simulink model "pvwindupfc11"  (R2016a)
settings: Solver=VariableStepAuto  StartTime=0.0  StopTime=0.5  RelTol=1e-3
undefined symbols (not defined in the file): BCMS11, c1, c2, c3, c4, c5, c6, Clink_3L, DiscIntNeverNeededParam, fdesignblkfcn, Fnom, gcbh, Ion, Ki_Ireg_3L, Ki_VDCreg_3L, Kp_Ireg_3L, Kp_VDCreg_3L, LimitL_Ireg_3L, LimitL_VDCreg_3L, LimitU_Ireg_3L, LimitU_VDCreg_3L, Lithium, LowerLimit, Pnom_3L, Pnom_dc_3L, PV11, Ts_Control, Ts_Power, Ts_PWM, UpperLimit, Vnom_dc_3L, Vnom_prim_3L, Vnom_sec_3L
libraries: powerlib x98, powerlib_extras x29, powerlib_meascontrol x20, fuzblock x2, simulink x1, electricdrivelib x1
(part 4 of 4)

== system pvwindupfc11/Control Systems /SEC Control/SEC Control System/Scaling ==
  Vdc : Inport
  VdVq : Inport  Port=2
  0.8 to 1.2 x Vnom_dc : Saturate  UpperLimit=1.5*Vnom_dc_3L  LowerLimit=0.5*Vnom_dc_3L
  Constant1 : Constant  Value=Vnom_sec_3L
  Gain1 : Gain  Gain=0.5/sqrt(2)*sqrt(3)
  Product : Product  Inputs=*/
  Product1 : Product  Inputs=**
  VdVq* : Outport
  wires:
  Product1/1 -> VdVq*/1
  VdVq/1 -> Product1/1
  Vdc/1 -> 0.8 to 1.2 x Vnom_dc/1
  Product/1 -> Product1/2
  0.8 to 1.2 x Vnom_dc/1 -> Gain1/1
  Gain1/1 -> Product/2
  Constant1/1 -> Product/1

== system pvwindupfc11/Control Systems /SEC Control/SEC Control System/VDC Controller ==
  Vdc : Inport  PortDimensions=1
  Vdc_ref : Inport  Port=2  PortDimensions=1
  Gain : Gain  Gain=1/(Vnom_dc_3L)
  PI_d : Subsystem  DialogController=POWERSYS.PowerSysDialog  mask(Discrete PI Controller){Kp=Kp_VDCreg_3L, Ki=Ki_VDCreg_3L, Par_Limits=[ LimitU_VDCreg_3L LimitL_VDCreg_3L ], Init=0, Ts=Ts_Control}
      mask prompts: Kp "Proportional gain (Kp):"; Ki "Integral gain (Ki):"; Par_Limits "Output limits: [ Upper   Lower ]"; Init "Output initial value:"; Ts "Sample time:"
      mask help: This block implements a discrete PI controller.
      mask init:
      | UpperLimit=Par_Limits(1);
      | LowerLimit=Par_Limits(2);
      mask Display: disp('PI');
  Sum : Sum  Inputs=|+-
  Idref : Outport
  wires:
  PI_d/1(Out) -> Idref/1
  Gain/1 -> PI_d/1(Error)
  Vdc/1 -> Sum/2
  Vdc_ref/1 -> Sum/1
  Sum/1 -> Gain/1

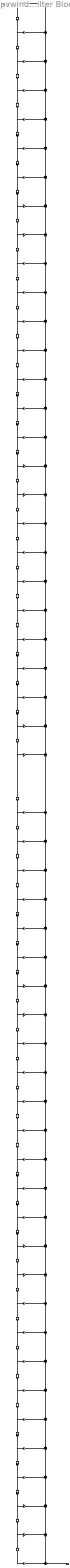
== system pvwindupfc11/Wind-MPPT/Torque reference 1/Differentiator Filter/Generated Filter Block ==
  Input : Inport
  BodyDelay{2..27,30..55} (52 alike) : Delay  DelayLength=1  InitialCondition=0  InputProcessing=Inherited
  BodyDelay29 : Delay  InitialCondition=0  InputProcessing=Inherited
  BodyLSum{2..27,29..55} (53 alike) : Sum  Inputs=++|  SaturateOnIntegerOverflow=on  InputSameDT=on  OutDataTypeStr=Inherit: Same as first input
  b(1) : Gain  Gain=0.0016485839041717864  SaturateOnIntegerOverflow=on  OutDataTypeStr=Inherit: Same as input  ParamDataTypeStr=Inherit: Same as input
  b(10) : Gain  Gain=0.011014879869749052  SaturateOnIntegerOverflow=on  OutDataTypeStr=Inherit: Same as input  ParamDataTypeStr=Inherit: Same as input
  b(11) : Gain  Gain=-0.005763535930488302  SaturateOnIntegerOverflow=on  OutDataTypeStr=Inherit: Same as input  ParamDataTypeStr=Inherit: Same as input
  b(12) : Gain  Gain=-0.0151981830555213  SaturateOnIntegerOverflow=on  OutDataTypeStr=Inherit: Same as input  ParamDataTypeStr=Inherit: Same as input
  b(13) : Gain  Gain=0.0065686388642668125  SaturateOnIntegerOverflow=on  OutDataTypeStr=Inherit: Same as input  ParamDataTypeStr=Inherit: Same as input
  b(14) : Gain  Gain=0.020867949959447688  SaturateOnIntegerOverflow=on  OutDataTypeStr=Inherit: Same as input  ParamDataTypeStr=Inherit: Same as input
  b(15) : Gain  Gain=-0.0070602627960907726  SaturateOnIntegerOverflow=on  OutDataTypeStr=Inherit: Same as input  ParamDataTypeStr=Inherit: Same as input
  b(16) : Gain  Gain=-0.028242635943863115  SaturateOnIntegerOverflow=on  OutDataTypeStr=Inherit: Same as input  ParamDataTypeStr=Inherit: Same as input
  b(17) : Gain  Gain=0.0072704924773104732  SaturateOnIntegerOverflow=on  OutDataTypeStr=Inherit: Same as input  ParamDataTypeStr=Inherit: Same as input
  b(18) : Gain  Gain=0.038329320446368831  SaturateOnIntegerOverflow=on  OutDataTypeStr=Inherit: Same as input  ParamDataTypeStr=Inherit: Same as input
  b(19) : Gain  Gain=-0.0068002265270407491  SaturateOnIntegerOverflow=on  OutDataTypeStr=Inherit: Same as input  ParamDataTypeStr=Inherit: Same as input
  b(2) : Gain  Gain=0.00017042943589110223  SaturateOnIntegerOverflow=on  OutDataTypeStr=Inherit: Same as input  ParamDataTypeStr=Inherit: Same as input
  b(20) : Gain  Gain=-0.052819993002155965  SaturateOnIntegerOverflow=on  OutDataTypeStr=Inherit: Same as input  ParamDataTypeStr=Inherit: Same as input
  b(21) : Gain  Gain=0.0049482783503700268  SaturateOnIntegerOverflow=on  OutDataTypeStr=Inherit: Same as input  ParamDataTypeStr=Inherit: Same as input
  b(22) : Gain  Gain=0.075871674298216826  SaturateOnIntegerOverflow=on  OutDataTypeStr=Inherit: Same as input  ParamDataTypeStr=Inherit: Same as input
  b(23) : Gain  Gain=0.00073312852370662537  SaturateOnIntegerOverflow=on  OutDataTypeStr=Inherit: Same as input  ParamDataTypeStr=Inherit: Same as input
  b(24) : Gain  Gain=-0.11992357305817197  SaturateOnIntegerOverflow=on  OutDataTypeStr=Inherit: Same as input  ParamDataTypeStr=Inherit: Same as input
  b(25) : Gain  Gain=-0.022982436984387535  SaturateOnIntegerOverflow=on  OutDataTypeStr=Inherit: Same as input  ParamDataTypeStr=Inherit: Same as input
  b(26) : Gain  Gain=0.24743192698089667  SaturateOnIntegerOverflow=on  OutDataTypeStr=Inherit: Same as input  ParamDataTypeStr=Inherit: Same as input
  b(27) : Gain  Gain=0.30572927022108953  SaturateOnIntegerOverflow=on  OutDataTypeStr=Inherit: Same as input  ParamDataTypeStr=Inherit: Same as input
  b(29) : Gain  Gain=-0.30572927022108953  SaturateOnIntegerOverflow=on  OutDataTypeStr=Inherit: Same as input  ParamDataTypeStr=Inherit: Same as input
  b(3) : Gain  Gain=-0.0038948238157296179  SaturateOnIntegerOverflow=on  OutDataTypeStr=Inherit: Same as input  ParamDataTypeStr=Inherit: Same as input
  b(30) : Gain  Gain=-0.24743192698089667  SaturateOnIntegerOverflow=on  OutDataTypeStr=Inherit: Same as input  ParamDataTypeStr=Inherit: Same as input
  b(31) : Gain  Gain=0.022982436984387535  SaturateOnIntegerOverflow=on  OutDataTypeStr=Inherit: Same as input  ParamDataTypeStr=Inherit: Same as input
  b(32) : Gain  Gain=0.11992357305817197  SaturateOnIntegerOverflow=on  OutDataTypeStr=Inherit: Same as input  ParamDataTypeStr=Inherit: Same as input
  b(33) : Gain  Gain=-0.00073312852370662537  SaturateOnIntegerOverflow=on  OutDataTypeStr=Inherit: Same as input  ParamDataTypeStr=Inherit: Same as input
  b(34) : Gain  Gain=-0.075871674298216826  SaturateOnIntegerOverflow=on  OutDataTypeStr=Inherit: Same as input  ParamDataTypeStr=Inherit: Same as input
  b(35) : Gain  Gain=-0.0049482783503700268  SaturateOnIntegerOverflow=on  OutDataTypeStr=Inherit: Same as input  ParamDataTypeStr=Inherit: Same as input
  b(36) : Gain  Gain=0.052819993002155965  SaturateOnIntegerOverflow=on  OutDataTypeStr=Inherit: Same as input  ParamDataTypeStr=Inherit: Same as input
  b(37) : Gain  Gain=0.0068002265270407491  SaturateOnIntegerOverflow=on  OutDataTypeStr=Inherit: Same as input  ParamDataTypeStr=Inherit: Same as input
  b(38) : Gain  Gain=-0.038329320446368831  SaturateOnIntegerOverflow=on  OutDataTypeStr=Inherit: Same as input  ParamDataTypeStr=Inherit: Same as input
  b(39) : Gain  Gain=-0.0072704924773104732  SaturateOnIntegerOverflow=on  OutDataTypeStr=Inherit: Same as input  ParamDataTypeStr=Inherit: Same as input
  b(4) : Gain  Gain=-0.0032830177673830877  SaturateOnIntegerOverflow=on  OutDataTypeStr=Inherit: Same as input  ParamDataTypeStr=Inherit: Same as input
  b(40) : Gain  Gain=0.028242635943863115  SaturateOnIntegerOverflow=on  OutDataTypeStr=Inherit: Same as input  ParamDataTypeStr=Inherit: Same as input
  b(41) : Gain  Gain=0.0070602627960907726  SaturateOnIntegerOverflow=on  OutDataTypeStr=Inherit: Same as input  ParamDataTypeStr=Inherit: Same as input
  b(42) : Gain  Gain=-0.020867949959447688  SaturateOnIntegerOverflow=on  OutDataTypeStr=Inherit: Same as input  ParamDataTypeStr=Inherit: Same as input
  b(43) : Gain  Gain=-0.0065686388642668125  SaturateOnIntegerOverflow=on  OutDataTypeStr=Inherit: Same as input  ParamDataTypeStr=Inherit: Same as input
  b(44) : Gain  Gain=0.0151981830555213  SaturateOnIntegerOverflow=on  OutDataTypeStr=Inherit: Same as input  ParamDataTypeStr=Inherit: Same as input
  b(45) : Gain  Gain=0.005763535930488302  SaturateOnIntegerOverflow=on  OutDataTypeStr=Inherit: Same as input  ParamDataTypeStr=Inherit: Same as input
  b(46) : Gain  Gain=-0.011014879869749052  SaturateOnIntegerOverflow=on  OutDataTypeStr=Inherit: Same as input  ParamDataTypeStr=Inherit: Same as input
  b(47) : Gain  Gain=-0.0051172092513206528  SaturateOnIntegerOverflow=on  OutDataTypeStr=Inherit: Same as input  ParamDataTypeStr=Inherit: Same as input
  b(48) : Gain  Gain=0.0075034408734532838  SaturateOnIntegerOverflow=on  OutDataTypeStr=Inherit: Same as input  ParamDataTypeStr=Inherit: Same as input
  b(49) : Gain  Gain=0.0039498824016694816  SaturateOnIntegerOverflow=on  OutDataTypeStr=Inherit: Same as input  ParamDataTypeStr=Inherit: Same as input
  b(5) : Gain  Gain=0.0039854203993547575  SaturateOnIntegerOverflow=on  OutDataTypeStr=Inherit: Same as input  ParamDataTypeStr=Inherit: Same as input
  b(50) : Gain  Gain=-0.0056185919166622817  SaturateOnIntegerOverflow=on  OutDataTypeStr=Inherit: Same as input  ParamDataTypeStr=Inherit: Same as input
  b(51) : Gain  Gain=-0.0039854203993547575  SaturateOnIntegerOverflow=on  OutDataTypeStr=Inherit: Same as input  ParamDataTypeStr=Inherit: Same as input
  b(52) : Gain  Gain=0.0032830177673830877  SaturateOnIntegerOverflow=on  OutDataTypeStr=Inherit: Same as input  ParamDataTypeStr=Inherit: Same as input
  b(53) : Gain  Gain=0.0038948238157296179  SaturateOnIntegerOverflow=on  OutDataTypeStr=Inherit: Same as input  ParamDataTypeStr=Inherit: Same as input
  b(54) : Gain  Gain=-0.00017042943589110223  SaturateOnIntegerOverflow=on  OutDataTypeStr=Inherit: Same as input  ParamDataTypeStr=Inherit: Same as input
  b(55) : Gain  Gain=-0.0016485839041717864  SaturateOnIntegerOverflow=on  OutDataTypeStr=Inherit: Same as input  ParamDataTypeStr=Inherit: Same as input
  b(6) : Gain  Gain=0.0056185919166622817  SaturateOnIntegerOverflow=on  OutDataTypeStr=Inherit: Same as input  ParamDataTypeStr=Inherit: Same as input
  b(7) : Gain  Gain=-0.0039498824016694816  SaturateOnIntegerOverflow=on  OutDataTypeStr=Inherit: Same as input  ParamDataTypeStr=Inherit: Same as input
  b(8) : Gain  Gain=-0.0075034408734532838  SaturateOnIntegerOverflow=on  OutDataTypeStr=Inherit: Same as input  ParamDataTypeStr=Inherit: Same as input
  b(9) : Gain  Gain=0.0051172092513206528  SaturateOnIntegerOverflow=on  OutDataTypeStr=Inherit: Same as input  ParamDataTypeStr=Inherit: Same as input
  Output : Outport
  wires:
  BodyLSum55/1 -> Output/1
  b(55)/1 -> BodyLSum55/2
  BodyDelay55/1 -> b(55)/1
  BodyLSum54/1 -> BodyLSum55/1
  b(54)/1 -> BodyLSum54/1
  BodyDelay54/1 -> BodyDelay55/1, b(54)/1
  BodyLSum53/1 -> BodyLSum54/2
  b(53)/1 -> BodyLSum53/1
  BodyDelay53/1 -> BodyDelay54/1, b(53)/1
  BodyLSum52/1 -> BodyLSum53/2
  b(52)/1 -> BodyLSum52/1
  BodyDelay52/1 -> BodyDelay53/1, b(52)/1
  BodyLSum51/1 -> BodyLSum52/2
  b(51)/1 -> BodyLSum51/1
  BodyDelay51/1 -> BodyDelay52/1, b(51)/1
  BodyLSum50/1 -> BodyLSum51/2
  b(50)/1 -> BodyLSum50/1
  BodyDelay50/1 -> BodyDelay51/1, b(50)/1
  BodyLSum49/1 -> BodyLSum50/2
  b(49)/1 -> BodyLSum49/1
  BodyDelay49/1 -> BodyDelay50/1, b(49)/1
  BodyLSum48/1 -> BodyLSum49/2
  b(48)/1 -> BodyLSum48/1
  BodyDelay48/1 -> BodyDelay49/1, b(48)/1
  BodyLSum47/1 -> BodyLSum48/2
  b(47)/1 -> BodyLSum47/1
  BodyDelay47/1 -> BodyDelay48/1, b(47)/1
  BodyLSum46/1 -> BodyLSum47/2
  b(46)/1 -> BodyLSum46/1
  BodyDelay46/1 -> BodyDelay47/1, b(46)/1
  BodyLSum45/1 -> BodyLSum46/2
  b(45)/1 -> BodyLSum45/1
  BodyDelay45/1 -> BodyDelay46/1, b(45)/1
  BodyLSum44/1 -> BodyLSum45/2
  b(44)/1 -> BodyLSum44/1
  BodyDelay44/1 -> BodyDelay45/1, b(44)/1
  BodyLSum43/1 -> BodyLSum44/2
  b(43)/1 -> BodyLSum43/1
  BodyDelay43/1 -> BodyDelay44/1, b(43)/1
  BodyLSum42/1 -> BodyLSum43/2
  b(42)/1 -> BodyLSum42/1
  BodyDelay42/1 -> BodyDelay43/1, b(42)/1
  BodyLSum41/1 -> BodyLSum42/2
  b(41)/1 -> BodyLSum41/1
  BodyDelay41/1 -> BodyDelay42/1, b(41)/1
  BodyLSum40/1 -> BodyLSum41/2
  b(40)/1 -> BodyLSum40/1
  BodyDelay40/1 -> BodyDelay41/1, b(40)/1
  BodyLSum39/1 -> BodyLSum40/2
  b(39)/1 -> BodyLSum39/1
  BodyDelay39/1 -> BodyDelay40/1, b(39)/1
  BodyLSum38/1 -> BodyLSum39/2
  b(38)/1 -> BodyLSum38/1
  BodyDelay38/1 -> BodyDelay39/1, b(38)/1
  BodyLSum37/1 -> BodyLSum38/2
  b(37)/1 -> BodyLSum37/1
  BodyDelay37/1 -> BodyDelay38/1, b(37)/1
  BodyLSum36/1 -> BodyLSum37/2
  b(36)/1 -> BodyLSum36/1
  BodyDelay36/1 -> BodyDelay37/1, b(36)/1
  BodyLSum35/1 -> BodyLSum36/2
  b(35)/1 -> BodyLSum35/1
  BodyDelay35/1 -> BodyDelay36/1, b(35)/1
  BodyLSum34/1 -> BodyLSum35/2
  b(34)/1 -> BodyLSum34/1
  BodyDelay34/1 -> BodyDelay35/1, b(34)/1
  BodyLSum33/1 -> BodyLSum34/2
  b(33)/1 -> BodyLSum33/1
  BodyDelay33/1 -> BodyDelay34/1, b(33)/1
  BodyLSum32/1 -> BodyLSum33/2
  b(32)/1 -> BodyLSum32/1
  BodyDelay32/1 -> BodyDelay33/1, b(32)/1
  BodyLSum31/1 -> BodyLSum32/2
  b(31)/1 -> BodyLSum31/1
  BodyDelay31/1 -> BodyDelay32/1, b(31)/1
  BodyLSum30/1 -> BodyLSum31/2
  b(30)/1 -> BodyLSum30/1
  BodyDelay30/1 -> BodyDelay31/1, b(30)/1
  BodyLSum29/1 -> BodyLSum30/2
  b(29)/1 -> BodyLSum29/1
  BodyDelay29/1 -> BodyDelay30/1, b(29)/1
  BodyLSum27/1 -> BodyLSum29/2
  b(27)/1 -> BodyLSum27/1
  BodyDelay27/1 -> BodyDelay29/1, b(27)/1
  BodyLSum26/1 -> BodyLSum27/2
  b(26)/1 -> BodyLSum26/1
  BodyDelay26/1 -> BodyDelay27/1, b(26)/1
  BodyLSum25/1 -> BodyLSum26/2
  b(25)/1 -> BodyLSum25/1
  BodyDelay25/1 -> BodyDelay26/1, b(25)/1
  BodyLSum24/1 -> BodyLSum25/2
  b(24)/1 -> BodyLSum24/1
  BodyDelay24/1 -> BodyDelay25/1, b(24)/1
  BodyLSum23/1 -> BodyLSum24/2
  b(23)/1 -> BodyLSum23/1
  BodyDelay23/1 -> BodyDelay24/1, b(23)/1
  BodyLSum22/1 -> BodyLSum23/2
  b(22)/1 -> BodyLSum22/1
  BodyDelay22/1 -> BodyDelay23/1, b(22)/1
  BodyLSum21/1 -> BodyLSum22/2
  b(21)/1 -> BodyLSum21/1
  BodyDelay21/1 -> BodyDelay22/1, b(21)/1
  BodyLSum20/1 -> BodyLSum21/2
  b(20)/1 -> BodyLSum20/1
  BodyDelay20/1 -> BodyDelay21/1, b(20)/1
  BodyLSum19/1 -> BodyLSum20/2
  b(19)/1 -> BodyLSum19/1
  BodyDelay19/1 -> BodyDelay20/1, b(19)/1
  BodyLSum18/1 -> BodyLSum19/2
  b(18)/1 -> BodyLSum18/1
  BodyDelay18/1 -> BodyDelay19/1, b(18)/1
  BodyLSum17/1 -> BodyLSum18/2
  b(17)/1 -> BodyLSum17/1
  BodyDelay17/1 -> BodyDelay18/1, b(17)/1
  BodyLSum16/1 -> BodyLSum17/2
  b(16)/1 -> BodyLSum16/1
  BodyDelay16/1 -> BodyDelay17/1, b(16)/1
  BodyLSum15/1 -> BodyLSum16/2
  b(15)/1 -> BodyLSum15/1
  BodyDelay15/1 -> BodyDelay16/1, b(15)/1
  BodyLSum14/1 -> BodyLSum15/2
  b(14)/1 -> BodyLSum14/1
  BodyDelay14/1 -> BodyDelay15/1, b(14)/1
  BodyLSum13/1 -> BodyLSum14/2
  b(13)/1 -> BodyLSum13/1
  BodyDelay13/1 -> BodyDelay14/1, b(13)/1
  BodyLSum12/1 -> BodyLSum13/2
  b(12)/1 -> BodyLSum12/1
  BodyDelay12/1 -> BodyDelay13/1, b(12)/1
  BodyLSum11/1 -> BodyLSum12/2
  b(11)/1 -> BodyLSum11/1
  BodyDelay11/1 -> BodyDelay12/1, b(11)/1
  BodyLSum10/1 -> BodyLSum11/2
  b(10)/1 -> BodyLSum10/1
  BodyDelay10/1 -> BodyDelay11/1, b(10)/1
  BodyLSum9/1 -> BodyLSum10/2
  b(9)/1 -> BodyLSum9/1
  BodyDelay9/1 -> BodyDelay10/1, b(9)/1
  BodyLSum8/1 -> BodyLSum9/2
  b(8)/1 -> BodyLSum8/1
  BodyDelay8/1 -> BodyDelay9/1, b(8)/1
  BodyLSum7/1 -> BodyLSum8/2
  b(7)/1 -> BodyLSum7/1
  BodyDelay7/1 -> BodyDelay8/1, b(7)/1
  BodyLSum6/1 -> BodyLSum7/2
  b(6)/1 -> BodyLSum6/1
  BodyDelay6/1 -> BodyDelay7/1, b(6)/1
  BodyLSum5/1 -> BodyLSum6/2
  b(5)/1 -> BodyLSum5/1
  BodyDelay5/1 -> BodyDelay6/1, b(5)/1
  BodyLSum4/1 -> BodyLSum5/2
  b(4)/1 -> BodyLSum4/1
  BodyDelay4/1 -> BodyDelay5/1, b(4)/1
  BodyLSum3/1 -> BodyLSum4/2
  b(3)/1 -> BodyLSum3/1
  BodyDelay3/1 -> BodyDelay4/1, b(3)/1
  BodyLSum2/1 -> BodyLSum3/2
  b(2)/1 -> BodyLSum2/1
  BodyDelay2/1 -> BodyDelay3/1, b(2)/1
  b(1)/1 -> BodyLSum2/2
  Input/1 -> BodyDelay2/1, b(1)/1

== system pvwindupfc11/Control Systems /SEC Control/SEC Control System/Current Controller/PI_d ==
  Error : Inport  SampleTime=Ts
  Discrete-Time Integrator : DiscreteIntegrator  InitialCondition=Init  SampleTime=Ts  LimitOutput=on  UpperSaturationLimit=UpperLimit  LowerSaturationLimit=LowerLimit  ICPrevOutput=DiscIntNeverNeededParam  ICPrevScaledInput=DiscIntNeverNeededParam
  Kp4 : Gain  Gain=Kp  SampleTime=Ts  SaturateOnIntegerOverflow=on  OutDataTypeStr=Inherit: Same as input  ParamDataTypeStr=Inherit: Same as input
  Kp5 : Gain  Gain=Ki  SampleTime=Ts  SaturateOnIntegerOverflow=on  OutDataTypeStr=Inherit: Same as input  ParamDataTypeStr=Inherit: Same as input
  Saturation2 : Saturate  UpperLimit=UpperLimit  LowerLimit=LowerLimit  SampleTime=Ts
  Sum6 : Sum  SampleTime=Ts  SaturateOnIntegerOverflow=on  InputSameDT=on  OutDataTypeStr=Inherit: Same as first input
  Zero-Order Hold : ZeroOrderHold  SampleTime=Ts
  Out : Outport  SampleTime=Ts  InitialOutput=0
  wires:
  Saturation2/1 -> Out/1
  Error/1 -> Kp4/1, Kp5/1
  Sum6/1 -> Saturation2/1
  Kp5/1 -> Discrete-Time Integrator/1
  Kp4/1 -> Zero-Order Hold/1
  Discrete-Time Integrator/1 -> Sum6/2
  Zero-Order Hold/1 -> Sum6/1

== system pvwindupfc11/Control Systems /SEC Control/SEC Control System/Current Controller/PI_q ==
  Error : Inport  SampleTime=Ts
  Discrete-Time Integrator : DiscreteIntegrator  InitialCondition=Init  SampleTime=Ts  LimitOutput=on  UpperSaturationLimit=UpperLimit  LowerSaturationLimit=LowerLimit  ICPrevOutput=DiscIntNeverNeededParam  ICPrevScaledInput=DiscIntNeverNeededParam
  Kp4 : Gain  Gain=Kp  SampleTime=Ts  SaturateOnIntegerOverflow=on  OutDataTypeStr=Inherit: Same as input  ParamDataTypeStr=Inherit: Same as input
  Kp5 : Gain  Gain=Ki  SampleTime=Ts  SaturateOnIntegerOverflow=on  OutDataTypeStr=Inherit: Same as input  ParamDataTypeStr=Inherit: Same as input
  Saturation2 : Saturate  UpperLimit=UpperLimit  LowerLimit=LowerLimit  SampleTime=Ts
  Sum6 : Sum  SampleTime=Ts  SaturateOnIntegerOverflow=on  InputSameDT=on  OutDataTypeStr=Inherit: Same as first input
  Zero-Order Hold : ZeroOrderHold  SampleTime=Ts
  Out : Outport  SampleTime=Ts  InitialOutput=0
  wires:
  Zero-Order Hold/1 -> Sum6/1
  Discrete-Time Integrator/1 -> Sum6/2
  Kp4/1 -> Zero-Order Hold/1
  Kp5/1 -> Discrete-Time Integrator/1
  Sum6/1 -> Saturation2/1
  Error/1 -> Kp5/1, Kp4/1
  Saturation2/1 -> Out/1

== system pvwindupfc11/Control Systems /SEC Control/SEC Control System/Current Controller/PQ ==
  ud : Inport
  id : Inport  Port=2
  uq : Inport  Port=3
  iq : Inport  Port=4
  Add : Sum
  Add1 : Sum  Inputs=+-
  Product{,1..3} (4 alike) : Product
  P : Outport
  Q : Outport  Port=2
  wires:
  id/1 -> Product2/2, Product/2
  Product/1 -> Add/1
  iq/1 -> Product3/1, Product1/2
  uq/1 -> Product2/1, Product1/1
  Product1/1 -> Add/2
  Add/1 -> P/1
  ud/1 -> Product3/2, Product/1
  Product2/1 -> Add1/1
  Product3/1 -> Add1/2
  Add1/1 -> Q/1

== system pvwindupfc11/Control Systems /SEC Control/SEC Control System/VDC Controller/PI_d ==
  Error : Inport  SampleTime=Ts
  Discrete-Time Integrator : DiscreteIntegrator  InitialCondition=Init  SampleTime=Ts  LimitOutput=on  UpperSaturationLimit=UpperLimit  LowerSaturationLimit=LowerLimit  ICPrevOutput=DiscIntNeverNeededParam  ICPrevScaledInput=DiscIntNeverNeededParam
  Kp4 : Gain  Gain=Kp  SampleTime=Ts  SaturateOnIntegerOverflow=on  OutDataTypeStr=Inherit: Same as input  ParamDataTypeStr=Inherit: Same as input
  Kp5 : Gain  Gain=Ki  SampleTime=Ts  SaturateOnIntegerOverflow=on  OutDataTypeStr=Inherit: Same as input  ParamDataTypeStr=Inherit: Same as input
  Saturation2 : Saturate  UpperLimit=UpperLimit  LowerLimit=LowerLimit  SampleTime=Ts
  Sum6 : Sum  SampleTime=Ts  SaturateOnIntegerOverflow=on  InputSameDT=on  OutDataTypeStr=Inherit: Same as first input
  Zero-Order Hold : ZeroOrderHold  SampleTime=Ts
  Out : Outport  SampleTime=Ts  InitialOutput=0
  wires:
  Saturation2/1 -> Out/1
  Error/1 -> Kp4/1, Kp5/1
  Sum6/1 -> Saturation2/1
  Kp5/1 -> Discrete-Time Integrator/1
  Kp4/1 -> Zero-Order Hold/1
  Discrete-Time Integrator/1 -> Sum6/2
  Zero-Order Hold/1 -> Sum6/1
